simulink model "pd_to_wheel_2"  (R2026a)
settings: Solver=ode45  StopTime=200  MaxStep=0.1
settings Model: Creator=user  LastModifiedBy=user

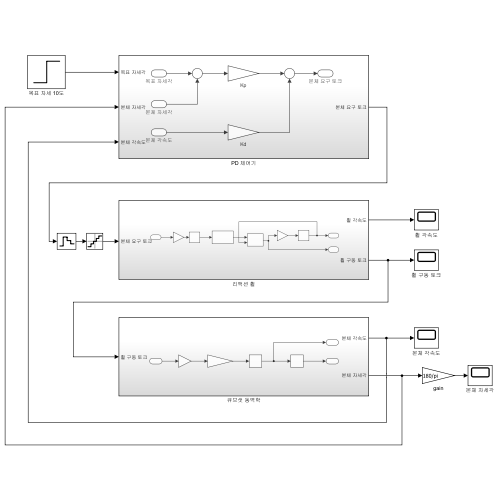
[thumbnail: Simulink's stored preview of the top-level diagram]
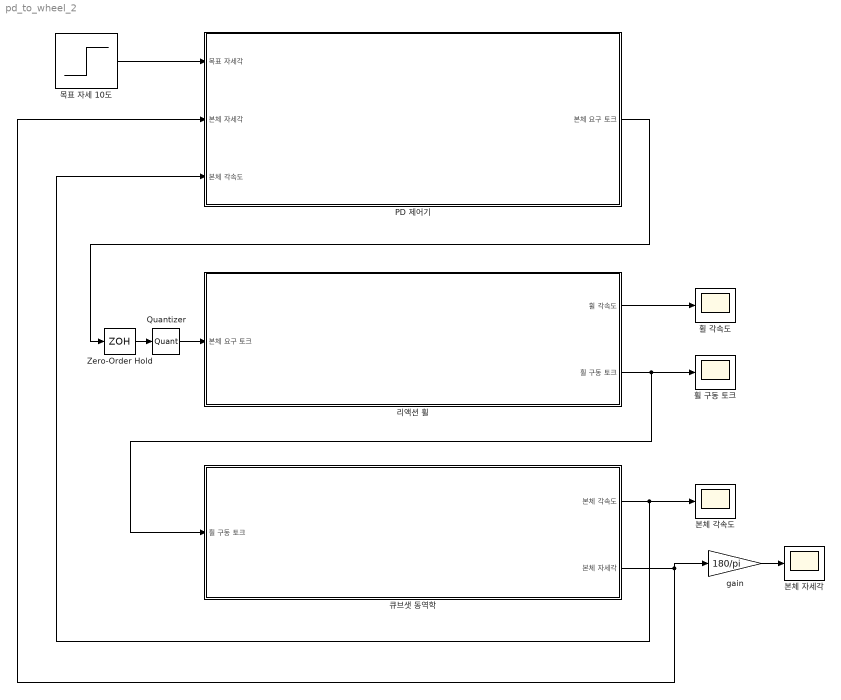
== system pd_to_wheel_2 ==
  PD 제어기 : Subsystem
  Quantizer : Quantizer  QuantizationInterval=1e-6
  Zero-Order Hold : ZeroOrderHold  SampleTime=0.2
  gain : Gain  Gain=180/pi
  리액션 휠 : Subsystem
  목표 자세 10도 : Step  FinalValue=10*pi/180  SampleTime=0
  본체 각속도 : Scope
      settings: ActiveDisplayYMinimum=-1  ActiveDisplayYMaximum=1  DataLoggingVariableName=ScopeData2
  본체 자세각 : Scope
      settings: ActiveDisplayYMinimum=-1  ActiveDisplayYMaximum=1
  큐브샛 동역학 : Subsystem
  휠 각속도 : Scope
      settings: ActiveDisplayYMinimum=-1  ActiveDisplayYMaximum=1
  휠 구동 토크 : Scope
      settings: ActiveDisplayYMinimum=-1  ActiveDisplayYMaximum=1  DataLoggingVariableName=ScopeData3
  wires:
  gain/1 -> 본체 자세각/1
  목표 자세 10도/1 -> PD 제어기/1(목표 자세각)
  큐브샛 동역학/1(본체 각속도) -> 본체 각속도/1, PD 제어기/3(본체 각속도)
  큐브샛 동역학/2(본체 자세각) -> PD 제어기/2(본체 자세각), gain/1
  리액션 휠/1(휠 각속도) -> 휠 각속도/1
  리액션 휠/2(휠 구동 토크) -> 휠 구동 토크/1, 큐브샛 동역학/1(휠 구동 토크)
  PD 제어기/1(본체 요구 토크) -> Zero-Order Hold/1
  Zero-Order Hold/1 -> Quantizer/1
  Quantizer/1 -> 리액션 휠/1(본체 요구 토크)

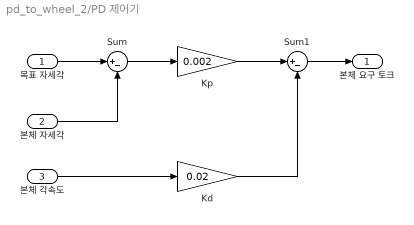
== system pd_to_wheel_2/PD 제어기 ==
  목표 자세각 : Inport
  본체 자세각 : Inport  Port=2
  본체 각속도 : Inport  Port=3
  Kd : Gain  Gain=0.02
  Kp : Gain  Gain=0.002
  Sum : Sum  Inputs=|+-
  Sum1 : Sum  Inputs=|+-
  본체 요구 토크 : Outport
  wires:
  Kd/1 -> Sum1/2
  Kp/1 -> Sum1/1
  본체 각속도/1 -> Kd/1
  Sum1/1 -> 본체 요구 토크/1
  Sum/1 -> Kp/1
  목표 자세각/1 -> Sum/1
  본체 자세각/1 -> Sum/2

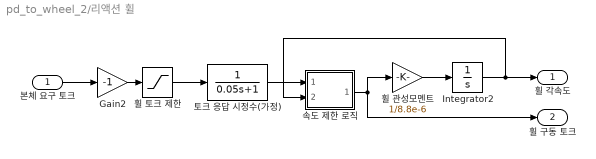
== system pd_to_wheel_2/리액션 휠 ==
  본체 요구 토크 : Inport
  Gain2 : Gain  Gain=-1
  Integrator2 : Integrator  LimitOutput=on  UpperSaturationLimit=6000*2*pi/60  LowerSaturationLimit=-6000*2*pi/60
  속도 제한 로직 : MATLAB Function  TreatAsAtomicUnit=on
  토크 응답 시정수(가정) : TransferFcn  Denominator=[0.05 1]
  휠 관성모멘트 : Gain  Gain=1/8.8e-6
  휠 토크 제한 : Saturate  UpperLimit=0.001  LowerLimit=-0.001
  휠 각속도 : Outport
  휠 구동 토크 : Outport  Port=2
  wires:
  본체 요구 토크/1 -> Gain2/1
  Integrator2/1 -> 속도 제한 로직/2(omega_w), 휠 각속도/1
  휠 관성모멘트/1 -> Integrator2/1
  Gain2/1 -> 휠 토크 제한/1
  속도 제한 로직/1(tau_out) -> 휠 구동 토크/1, 휠 관성모멘트/1
  휠 토크 제한/1 -> 토크 응답 시정수(가정)/1
  토크 응답 시정수(가정)/1 -> 속도 제한 로직/1(tau_in)

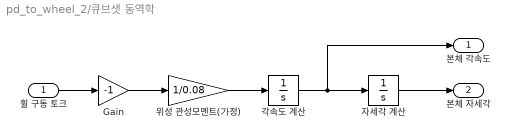
== system pd_to_wheel_2/큐브샛 동역학 ==
  휠 구동 토크 : Inport
  Gain : Gain  Gain=-1
  각속도 계산 : Integrator
  위성 관성모멘트(가정) : Gain  Gain=1/0.08
  자세각 계산 : Integrator
  본체 각속도 : Outport
  본체 자세각 : Outport  Port=2
  wires:
  위성 관성모멘트(가정)/1 -> 각속도 계산/1
  Gain/1 -> 위성 관성모멘트(가정)/1
  각속도 계산/1 -> 본체 각속도/1, 자세각 계산/1
  휠 구동 토크/1 -> Gain/1
  자세각 계산/1 -> 본체 자세각/1

== matlab function pd_to_wheel_2/리액션 휠/속도 제한 로직 ==
  data: tau_in input; tau_out output; omega_w input
function tau_out = wheel_speed_limit(tau_in, omega_w)
% Wheel speed saturation test
% tau_in  : Wheel torque [Nm]
% omega_w : Wheel angular velocity [rad/s]

omega_max = 6000 * 2*pi / 60;

tau_out = tau_in;

if omega_w >= omega_max && tau_in > 0
    tau_out = 0;
elseif omega_w <= -omega_max && tau_in < 0
    tau_out = 0;
end
end
